simulink model "FrameTrackingPITest"  (R2026b)
settings: Solver=FixedStepDiscrete  StopTime=testCfg.StopTime  FixedStep=currentCfg.Ts
PostLoadFcn:
  | addpath(fullfile(fileparts(get_param(bdroot,'FileName')),'..','build_process'));initialize_frame_pi_test(bdroot);
model workspace (MAT data in the model file):
  currentCfg.Ts = 5e-05
  currentCfg.BandwidthHz = 500
  currentCfg.Kpd = 3.14159265359
  currentCfg.Kpq = 3.76991118431
  currentCfg.Kid = 1570.79632679
  currentCfg.Kiq = 1570.79632679
  currentCfg.Kaw = 1000
  inverterCfg.Vdc = 48
  inverterCfg.MinDuty = 0.02
  inverterCfg.PwmTs = 0.0001
  inverterCfg.LinearLimit = 26.6043004043
  testCfg.UseInternalLimit = 0
  testCfg.StopTime = 0.06
  testStim.time = [0 5e-05 0.0001 0.00015 0.0002 0.00025 0.0003 0.00035 0.0004 0.00045 0.0005 0.00055 ... (1201 elements, 1201x1)]
  testStim.signals.values = [0.2 0.2 0.2 0.2 0.2 0.2 0.2 0.2 0.2 0.2 0.2 0.2 ... (12010 elements, 1201x10)]
  testStim.signals.dimensions = 10
libraries: CurrentControl x3
settings Model: Creator=24322  LastModifiedBy=24322

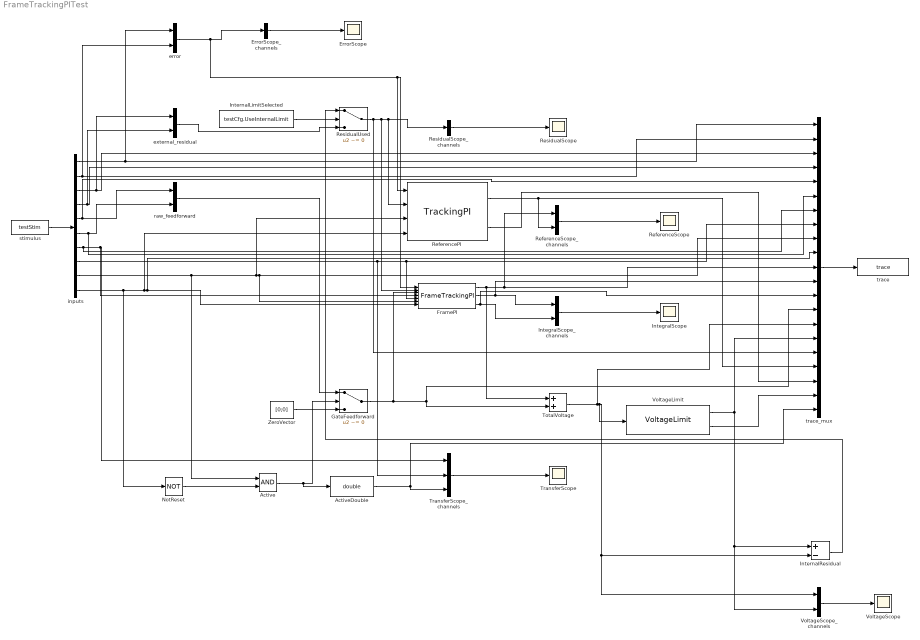
== system FrameTrackingPITest ==
  Active : Logic  IconShape=distinctive  AllPortsSameDT=off  OutDataTypeStr=boolean
  ActiveDouble : DataTypeConversion  OutDataTypeStr=double  SaturateOnIntegerOverflow=off  RndMeth=Floor
  ErrorScope : Scope
  ErrorScope_channels : Mux  Inputs=1
  FramePI : CurrentControl/FrameTrackingPI  currentCfg=currentCfg
  GateFeedforward : Switch  Criteria=u2 ~= 0  SaturateOnIntegerOverflow=off  InputSameDT=off
  IntegralScope : Scope
  IntegralScope_channels : Mux  Inputs=2
  InternalLimitSelected : Constant  Value=testCfg.UseInternalLimit
  InternalResidual : Sum  Inputs=+-
  NotReset : Logic  Operator=NOT  Inputs=1  IconShape=distinctive  AllPortsSameDT=off  OutDataTypeStr=boolean
  ReferencePI : CurrentControl/TrackingPI  SystemSampleTime=-1  VariantActivationTime=update diagram  EmptyChoice=off  PassThrough=off  PassThroughVariantControl=(default)  EmptyChoiceVariantControl=(default)  AllowFlexibleInterface=on  Latency=0  AutoFrameSizeCalculation=off
  ReferenceScope : Scope
  ReferenceScope_channels : Mux  Inputs=2
  ResidualScope : Scope
  ResidualScope_channels : Mux  Inputs=1
  ResidualUsed : Switch  Criteria=u2 ~= 0  SaturateOnIntegerOverflow=off  InputSameDT=off
  TotalVoltage : Sum
  TransferScope : Scope
  TransferScope_channels : Mux  Inputs=3
  VoltageLimit : CurrentControl/VoltageLimit  SystemSampleTime=-1  VariantActivationTime=update diagram  EmptyChoice=off  PassThrough=off  PassThroughVariantControl=(default)  EmptyChoiceVariantControl=(default)  AllowFlexibleInterface=on  Latency=0  AutoFrameSizeCalculation=off
  VoltageScope : Scope
  VoltageScope_channels : Mux  Inputs=2
  ZeroVector : Constant  Value=[0;0]
  error : Mux  Inputs=2
  external_residual : Mux  Inputs=2
  inputs : Demux  Outputs=10
  raw_feedforward : Mux  Inputs=2
  stimulus : FromWorkspace  VariableName=testStim  SampleTime=currentCfg.Ts  Interpolate=off  OutputAfterFinalValue=Holding final value
  trace : ToWorkspace  VariableName=trace  SaveFormat=Structure With Time  SampleTime=-1
  trace_mux : Mux  Inputs=21
  wires:
  TransferScope_channels/1 -> TransferScope/1
  ReferenceScope_channels/1 -> ReferenceScope/1
  ResidualScope_channels/1 -> ResidualScope/1
  IntegralScope_channels/1 -> IntegralScope/1
  VoltageScope_channels/1 -> VoltageScope/1
  ErrorScope_channels/1 -> ErrorScope/1
  ActiveDouble/1 -> trace_mux/21, TransferScope_channels/3
  VoltageLimit/2 -> trace_mux/20
  ReferencePI/2 -> trace_mux/19
  ReferencePI/1 -> trace_mux/18, ReferenceScope_channels/2
  FramePI/3 -> trace_mux/13, IntegralScope_channels/2
  FramePI/2 -> trace_mux/12, IntegralScope_channels/1
  external_residual/1 -> ResidualUsed/3
  InternalLimitSelected/1 -> ResidualUsed/2
  InternalResidual/1 -> ResidualUsed/1
  VoltageLimit/1 -> InternalResidual/1, VoltageScope_channels/2, trace_mux/16
  TotalVoltage/1 -> InternalResidual/2, VoltageScope_channels/1, VoltageLimit/1, trace_mux/15
  FramePI/1 -> trace_mux/11, ReferenceScope_channels/1, TotalVoltage/1
  inputs/8 -> FramePI/5, trace_mux/8, TransferScope_channels/2
  inputs/7 -> FramePI/4, TransferScope_channels/1, trace_mux/7
  GateFeedforward/1 -> TotalVoltage/2, trace_mux/14, FramePI/3
  ResidualUsed/1 -> ResidualScope_channels/1, ReferencePI/2, FramePI/2, trace_mux/17
  error/1 -> FramePI/1, ReferencePI/1, ErrorScope_channels/1
  ZeroVector/1 -> GateFeedforward/3
  raw_feedforward/1 -> GateFeedforward/1
  Active/1 -> GateFeedforward/2, ActiveDouble/1
  NotReset/1 -> Active/2
  inputs/9 -> trace_mux/9, FramePI/6, ReferencePI/3, Active/1
  inputs/10 -> FramePI/7, trace_mux/10, ReferencePI/4, NotReset/1
  inputs/6 -> raw_feedforward/2, trace_mux/6
  inputs/5 -> raw_feedforward/1, trace_mux/5
  inputs/4 -> external_residual/2, trace_mux/4
  inputs/3 -> external_residual/1, trace_mux/3
  inputs/2 -> error/2, trace_mux/2
  inputs/1 -> error/1, trace_mux/1
  trace_mux/1 -> trace/1
  stimulus/1 -> inputs/1
